simulink model "DR_ScreeningResourceModel"  (R2025b)
settings: Solver=VariableStepAuto  StartTime=0.0  StopTime=24  RelTol=1e-3
settings Model: Creator=Nitin Kumar Shukla  LastModifiedBy=Nitin Kumar Shukla

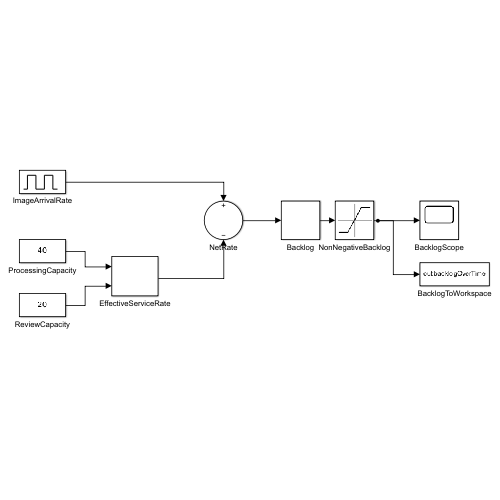
[thumbnail: Simulink's stored preview of the top-level diagram]
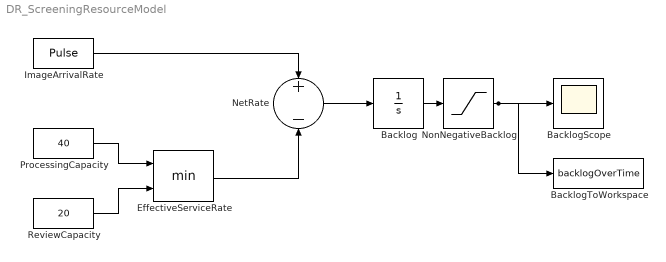
== system DR_ScreeningResourceModel ==
  Backlog : Integrator
  BacklogScope : Scope
  BacklogToWorkspace : ToWorkspace  VariableName=backlogOverTime  SaveFormat=Timeseries  SampleTime=-1
  EffectiveServiceRate : MinMax  Inputs=2
  ImageArrivalRate : DiscretePulseGenerator  PulseType=Time based  Amplitude=15  Period=1  PulseWidth=60
  NetRate : Sum  Inputs=+-
  NonNegativeBacklog : Saturate  UpperLimit=inf  LowerLimit=0
  ProcessingCapacity : Constant  Value=40
  ReviewCapacity : Constant  Value=20
  wires:
  ProcessingCapacity/1 -> EffectiveServiceRate/1
  ReviewCapacity/1 -> EffectiveServiceRate/2
  ImageArrivalRate/1 -> NetRate/1
  EffectiveServiceRate/1 -> NetRate/2
  NetRate/1 -> Backlog/1
  Backlog/1 -> NonNegativeBacklog/1
  NonNegativeBacklog/1 -> BacklogScope/1, BacklogToWorkspace/1
